simulink model "OpenLoop_2step"  (R2025a)
settings: Solver=ode4  StartTime=0.0  StopTime=5250  FixedStep=DT  MaxStep=DT  RelTol=1e-3  EnableMultiTasking=on
values from neighbouring files (symbols this model uses):
  particion = 301    [Run_OpenLoop_pr_2step.m]    (also in Run_OpenLoop_tl_2step.m)
  Ts = 0.025    [Run_OpenLoop_pr_2step.m]    (also in Run_OpenLoop_tl_2step.m)
  zona = 0.09    [Run_OpenLoop_pr_2step.m]    (also in Run_OpenLoop_tl_2step.m)
undefined symbols (not defined in the file or in its folder): DiscIntNeverNeededParam, OutList, strmatch
libraries: rllib x1
settings Model: Creator=bjonkman  LastModifiedBy=celop
settings SolverCC: AlgebraicLoopSolver=TrustRegion  AutoInsertRateTranBlk=on
settings DataIOCC: LimitDataPoints=on  SaveFormat=Array  SignalLoggingSaveFormat=ModelDataLogs  SaveOutput=off  SaveTime=off  SignalLoggingName=sigsOut
settings OptimizationCC: ExpressionDepthLimit=2147483647.0  LifeSpan=inf
settings DebuggingCC: SaveWithParameterizedLinksMsg=none  UnderspecifiedInitializationDetection=Classic  MergeDetectMultiDrivingBlocksExec=none  SignalResolutionControl=TryResolveAllWithWarning  MultiTaskDSMMsg=warning  MultiTaskCondExecSysMsg=none  FcnCallInpInsideContextMsg=warning  UnconnectedInputMsg=warning  UnconnectedOutputMsg=warning  UnconnectedLineMsg=warning  StateNameClashWarn=warning  SFUnexpectedBacktrackingDiag=warning  SFNoUnconditionalDefaultTransitionDiag=warning  SFExecutionAtInitializationDiag=none  ArithmeticOperatorsInVariantConditions=warning
settings HardwareCC: ProdBitPerPointer=32.0  ProdBitPerSizeT=32.0  ProdBitPerPtrDiffT=32.0  ProdLargestAtomicFloat=None  ProdIntDivRoundTo=Undefined  ProdEndianess=Unspecified  ProdWordSize=32.0  ProdHWDeviceType=32-bit Generic  TargetUnknown=on
settings ModelReferenceCC: EnableRefExpFcnMdlSchedulingChecks=on  PropagateSignalLabelsOutOfModel=off
settings SFSimCC: SimUseLocalCustomCode=off  CustomCodeUndefinedFunction=UseInterfaceOnly
settings RTWCC: RTWUseLocalCustomCode=off  GPUComputeCapability=3.5  DLArmComputeVersion=19.05
settings CodeAppCC: StateflowObjectComments=on
settings GRTTargetCC: TargetLangStandard=C89/C90 (ANSI)  CombineOutputUpdateFcns=off  GRTInterface=on
settings ConfigComp: CovMetricSettings=dw  CovSaveCumulativeToWorkspaceVar=on  CovSaveSingleToWorkspaceVar=on  CovExternalEMLEnable=off

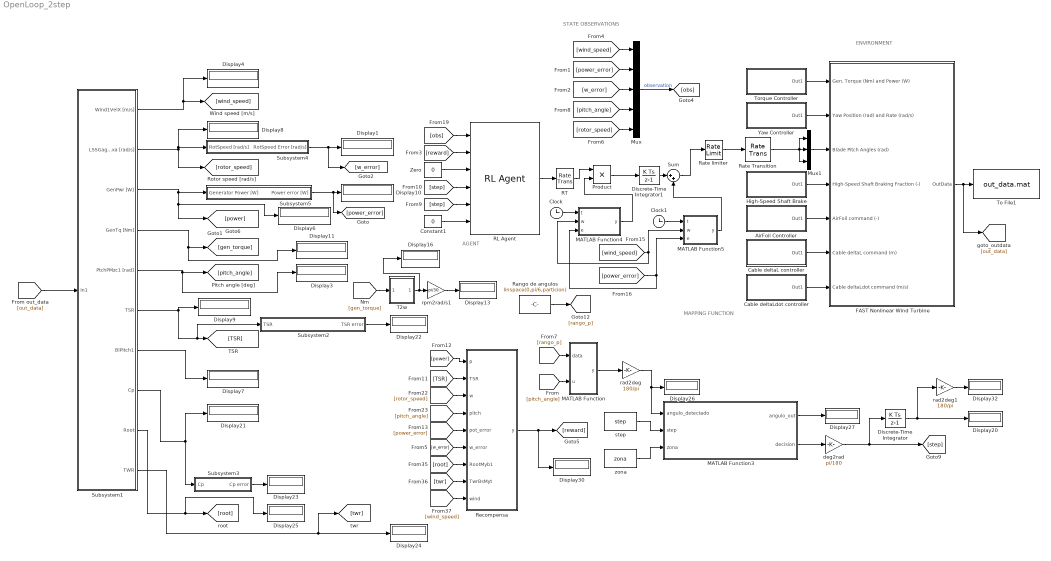
== system OpenLoop_2step ==
  note: STATE OBSERVATIONS
  note: AGENT
  note: ENVIRONMENT
  note: MAPPING FUNCTION
  AirFoil Controller : Subsystem
  Cable deltaL controller : Subsystem
  Cable deltaLdot controller : Subsystem
  Clock : Clock
  Clock1 : Clock
  Constant1 : Constant  Value=0
  Discrete-Time Integrator : DiscreteIntegrator  gainval=1.0/Ts  SampleTime=Ts  LimitOutput=on  UpperSaturationLimit=pi/6  LowerSaturationLimit=0  ICPrevOutput=DiscIntNeverNeededParam  ICPrevScaledInput=DiscIntNeverNeededParam
  Discrete-Time Integrator1 : DiscreteIntegrator  gainval=1.0/Ts  SampleTime=Ts  LimitOutput=on  UpperSaturationLimit=pi/6  LowerSaturationLimit=0  ICPrevOutput=DiscIntNeverNeededParam  ICPrevScaledInput=DiscIntNeverNeededParam
  Display{1,3..4,6..11,13,16,20..27,30,32} (21 alike) : Display
      Display30 settings: Format=short_e
  FAST Nonlinear Wind Turbine : Subsystem  mask(FAST Nonlinear Wind Turbine){}
      mask help: This block contains the FAST S-Function.
      mask init:
      | clear FAST_SFunc
  High-Speed Shaft Brake : Subsystem
  MATLAB Function : MATLAB Function  TreatAsAtomicUnit=on
  MATLAB Function3 : MATLAB Function  TreatAsAtomicUnit=on
  MATLAB Function4 : MATLAB Function  TreatAsAtomicUnit=on
  MATLAB Function5 : MATLAB Function  TreatAsAtomicUnit=on
  Mux : Mux  Inputs=5
  Mux1 : Mux  Inputs=3
  Product : Product
  RL Agent : rllib/RL Agent  Agent=agent  ExternalActionAsInput=on  ProvideLastAction=on  ProvideCumRwd=off  TreatAsDirectFeedthrough=on  UseStrictObservationDataTypes=off
  RT : RateTransition  OutPortSampleTime=0.025
  Rango de angulos : Constant  Value=linspace(0,pi/6,particion)
  Rate Transition : RateTransition  OutPortSampleTime=0.025
  Rate limiter : RateLimiter  RisingSlewLimit=7*pi/180  FallingSlewLimit=-7*pi/180  LinearizeAsGain=off
  Recompensa : MATLAB Function  TreatAsAtomicUnit=on
  Subsystem1 : Subsystem
  Subsystem2 : Subsystem
  Subsystem3 : Subsystem
  Subsystem4 : Subsystem
  Subsystem5 : Subsystem
  Sum : Sum  Inputs=|++
  T2w : Subsystem
  To File1 : ToFile  Filename=out_data.mat  MatrixName=data
  Torque Controller : Subsystem
  Yaw Controller : Subsystem
  Zero : Constant  Value=0  OutDataTypeStr=Inherit: Inherit via back propagation
  deg2rad : Gain  Gain=pi/180
  rad2deg : Gain  Gain=180/pi
  rad2deg1 : Gain  Gain=180/pi
  rpm2rad/s1 : Gain  Gain=pi/30
  step : Constant  Value=step
  zona : Constant  Value=zona
  wires:
  Yaw Controller/1(Out1) -> FAST Nonlinear Wind Turbine/2(Yaw Position (rad) and Rate (rad/s))
  High-Speed Shaft Brake/1(Out1) -> FAST Nonlinear Wind Turbine/4(High-Speed Shaft Braking Fraction (-))
  AirFoil Controller/1(Out1) -> FAST Nonlinear Wind Turbine/5(AirFoil command (-))
  Cable deltaL controller/1(Out1) -> FAST Nonlinear Wind Turbine/6(Cable deltaL command (m))
  Cable deltaLdot controller/1(Out1) -> FAST Nonlinear Wind Turbine/7(Cable deltaLdot command (m/s))
  Zero/1 -> RL Agent/3
  [rango_p] -> MATLAB Function/1(data)
  FAST Nonlinear Wind Turbine/1(OutData) -> To File1/1, [out_data]
  [out_data] -> Subsystem1/1(In1)
  Rate Transition/1 -> Mux1/3, Mux1/1, Mux1/2
  Constant1/1 -> RL Agent/6
  Subsystem1/3(GenPwr [W]) -> [power], Display6/1, Subsystem5/1(Generator Power [W])
  Subsystem1/1(Wind1VelX [m/s]) -> Display4/1, [wind_speed]
  Subsystem1/2(LSSGagVxa [rad/s]) -> Display8/1, Subsystem4/1(RotSpeed [rad/s]), [rotor_speed]
  [pitch_angle] -> MATLAB Function/2(u)
  [wind_speed] -> Mux/1
  MATLAB Function/1(y) -> rad2deg/1
  Subsystem1/5(PtchPMzc1 [rad]) -> Display3/1, [pitch_angle]
  Recompensa/1(y) -> Display30/1, [reward]
  [TSR] -> Recompensa/2(TSR)
  [pitch_angle] -> Recompensa/4(pitch)
  [rotor_speed] -> Recompensa/3(w)
  [power] -> Recompensa/1(p)
  Subsystem1/6(TSR) -> Display9/1, Subsystem2/1(TSR), [TSR]
  [power_error] -> Recompensa/5(pot_error)
  Subsystem1/7(BlPitch1) -> Display7/1
  [power_error] -> Mux/2
  [rotor_speed] -> Mux/5
  [pitch_angle] -> Mux/4
  [w_error] -> Mux/3
  [w_error] -> Recompensa/6(w_error)
  Rango de angulos/1 -> [rango_p]
  Subsystem5/1(Power error [W]) -> Display10/1, [power_error]
  Subsystem1/4(GenTq [Nm]) -> Display11/1, [gen_torque]
  Subsystem4/1(RotSpeed Error [rad/s]) -> Display1/1, [w_error]
  [gen_torque] -> T2w/1(In1)
  Mux/1 -> [obs]  "observation"
  [obs] -> RL Agent/1
  rpm2rad/s1/1 -> Display13/1
  T2w/1(Out1) -> Display16/1, rpm2rad/s1/1
  Subsystem2/1(TSR error) -> Display22/1
  Mux1/1 -> FAST Nonlinear Wind Turbine/3(Blade Pitch Angles (rad))
  Subsystem1/8(Cp) -> Subsystem3/1(Cp), Display21/1
  Subsystem3/1(Cp error) -> Display23/1
  [reward] -> RL Agent/2
  [root] -> Recompensa/7(RootMyb1)
  [twr] -> Recompensa/8(TwrBsMyt)
  Subsystem1/10(TWR) -> Display24/1, [twr]
  Subsystem1/9(Root) -> Display25/1, [root]
  rad2deg/1 -> Display26/1, MATLAB Function3/1(angulo_detectado)
  MATLAB Function3/1(angulo_out) -> Display27/1
  MATLAB Function3/2(decision) -> deg2rad/1
  [wind_speed] -> Recompensa/9(wind)
  Discrete-Time Integrator/1 -> rad2deg1/1, Display20/1
  rad2deg1/1 -> Display32/1
  [step] -> RL Agent/5
  [step] -> RL Agent/4
  deg2rad/1 -> [step], Discrete-Time Integrator/1
  step/1 -> MATLAB Function3/2(step)
  zona/1 -> MATLAB Function3/3(zona)
  Clock/1 -> MATLAB Function4/1(t)
  MATLAB Function4/1(y) -> Product/2
  [wind_speed] -> MATLAB Function4/2(w), MATLAB Function5/2(w)
  Product/1 -> Discrete-Time Integrator1/1
  RL Agent/1 -> RT/1
  Rate limiter/1 -> Rate Transition/1
  [power_error] -> MATLAB Function5/3(e), MATLAB Function4/3(e)
  RT/1 -> Product/1
  Discrete-Time Integrator1/1 -> Sum/1
  Sum/1 -> Rate limiter/1
  Clock1/1 -> MATLAB Function5/1(t)
  MATLAB Function5/1(y) -> Sum/2
  Torque Controller/1(Out1) -> FAST Nonlinear Wind Turbine/1(Gen. Torque (Nm) and Power (W))

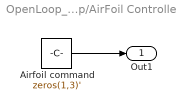
== system OpenLoop_2step/AirFoil Controller ==
  Airfoil command : Constant  Value=zeros(1,3)'
  Out1 : Outport
  wires:
  Airfoil command/1 -> Out1/1

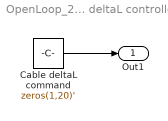
== system OpenLoop_2step/Cable deltaL controller ==
  Cable deltaL command : Constant  Value=zeros(1,20)'
  Out1 : Outport
  wires:
  Cable deltaL command/1 -> Out1/1

== system OpenLoop_2step/Cable deltaLdot controller ==
  Cable deltaLdot command : Constant  Value=zeros(1,20)'
  Out1 : Outport
  wires:
  Cable deltaLdot command/1 -> Out1/1

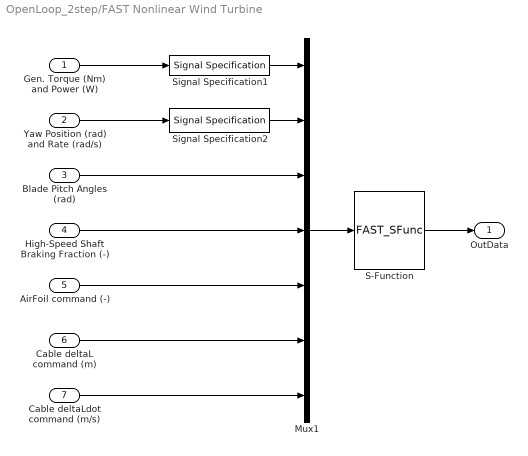
== system OpenLoop_2step/FAST Nonlinear Wind Turbine ==
  Gen. Torque (Nm) and Power (W) : Inport
  Yaw Position (rad) and Rate (rad/s) : Inport  Port=2
  Blade Pitch Angles (rad) : Inport  Port=3
  High-Speed Shaft Braking Fraction (-) : Inport  Port=4
  AirFoil command (-) : Inport  Port=5
  Cable deltaL command (m) : Inport  Port=6
  Cable deltaLdot command (m/s) : Inport  Port=7
  Mux1 : Mux  Inputs=7
  S-Function : S-Function  FunctionName=FAST_SFunc  Parameters=FAST_InputFileName, TMax, 0  SFunctionDeploymentMode=off  EnableBusSupport=off
  Signal Specification1 : SignalSpecification  OutDataTypeStr=double  Dimensions=2
  Signal Specification2 : SignalSpecification  OutDataTypeStr=double  Dimensions=2
  OutData : Outport
  wires:
  Gen. Torque (Nm) and Power (W)/1 -> Signal Specification1/1
  S-Function/1 -> OutData/1
  Mux1/1 -> S-Function/1
  Blade Pitch Angles (rad)/1 -> Mux1/3
  Yaw Position (rad) and Rate (rad/s)/1 -> Signal Specification2/1
  Signal Specification1/1 -> Mux1/1
  Signal Specification2/1 -> Mux1/2
  High-Speed Shaft Braking Fraction (-)/1 -> Mux1/4
  AirFoil command (-)/1 -> Mux1/5
  Cable deltaL command (m)/1 -> Mux1/6
  Cable deltaLdot command (m/s)/1 -> Mux1/7

== system OpenLoop_2step/High-Speed Shaft Brake ==
  High-Speed Shaft Braking Fraction : Constant  Value=0
  Out1 : Outport
  wires:
  High-Speed Shaft Braking Fraction/1 -> Out1/1

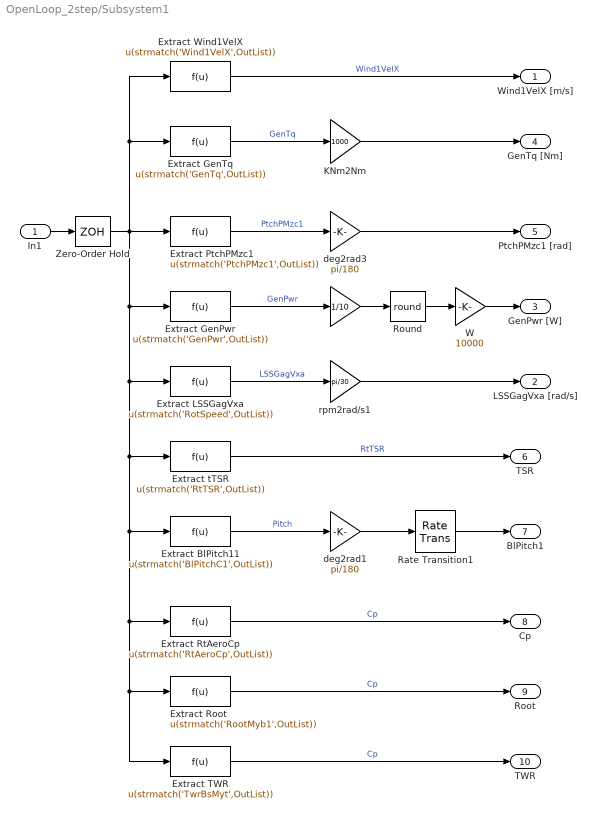
== system OpenLoop_2step/Subsystem1 ==
  In1 : Inport
  " " : Gain  Gain=1/10
  Extract BlPitch11 : Fcn  Expr=u(strmatch('BlPitchC1',OutList))
  Extract GenPwr : Fcn  Expr=u(strmatch('GenPwr',OutList))
  Extract GenTq : Fcn  Expr=u(strmatch('GenTq',OutList))
  Extract LSSGagVxa : Fcn  Expr=u(strmatch('RotSpeed',OutList))
  Extract PtchPMzc1 : Fcn  Expr=u(strmatch('PtchPMzc1',OutList))
  Extract Root : Fcn  Expr=u(strmatch('RootMyb1',OutList))
  Extract RtAeroCp : Fcn  Expr=u(strmatch('RtAeroCp',OutList))
  Extract TWR : Fcn  Expr=u(strmatch('TwrBsMyt',OutList))
  Extract Wind1VelX : Fcn  Expr=u(strmatch('Wind1VelX',OutList))
  Extract tTSR : Fcn  Expr=u(strmatch('RtTSR',OutList))
  KNm2Nm : Gain  Gain=1000
  Rate Transition1 : RateTransition  OutPortSampleTime=Ts
  Round : Rounding  Operator=round
  W : Gain  Gain=10000
  Zero-Order Hold : ZeroOrderHold  SampleTime=Ts
  deg2rad1 : Gain  Gain=pi/180
  deg2rad3 : Gain  Gain=pi/180
  rpm2rad/s1 : Gain  Gain=pi/30
  Wind1VelX [m/s] : Outport
  LSSGagVxa [rad/s] : Outport  Port=2
  GenPwr [W] : Outport  Port=3
  GenTq [Nm] : Outport  Port=4
  PtchPMzc1 [rad] : Outport  Port=5
  TSR : Outport  Port=6
  BlPitch1 : Outport  Port=7
  Cp : Outport  Port=8
  Root : Outport  Port=9
  TWR : Outport  Port=10
  wires:
  KNm2Nm/1 -> GenTq [Nm]/1
  Extract GenTq/1 -> KNm2Nm/1  "GenTq"
  Extract Wind1VelX/1 -> Wind1VelX [m/s]/1  "Wind1VelX"
  deg2rad3/1 -> PtchPMzc1 [rad]/1
  Extract PtchPMzc1/1 -> deg2rad3/1  "PtchPMzc1"
  Extract LSSGagVxa/1 -> rpm2rad/s1/1  "LSSGagVxa"
  Extract GenPwr/1 -> " "/1  "GenPwr"
  rpm2rad/s1/1 -> LSSGagVxa [rad/s]/1
  W/1 -> GenPwr [W]/1
  " "/1 -> Round/1
  Round/1 -> W/1
  In1/1 -> Zero-Order Hold/1
  Zero-Order Hold/1 -> Extract BlPitch11/1, Extract RtAeroCp/1, Extract Root/1, Extract TWR/1, Extract tTSR/1, Extract LSSGagVxa/1, Extract GenPwr/1, Extract GenTq/1, Extract Wind1VelX/1, Extract PtchPMzc1/1
  Extract tTSR/1 -> TSR/1  "RtTSR"
  Extract BlPitch11/1 -> deg2rad1/1  "Pitch"
  deg2rad1/1 -> Rate Transition1/1
  Rate Transition1/1 -> BlPitch1/1
  Extract RtAeroCp/1 -> Cp/1  "Cp"
  Extract TWR/1 -> TWR/1  "Cp"
  Extract Root/1 -> Root/1  "Cp"

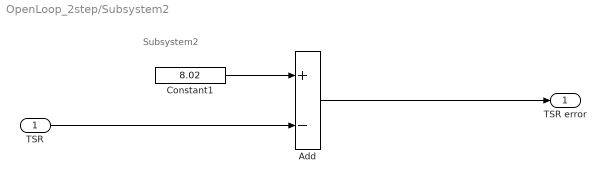
== system OpenLoop_2step/Subsystem2 ==
  note: Subsystem2
  TSR : Inport
  Add : Sum  Inputs=+-
  Constant1 : Constant  Value=8.02  SampleTime=Ts
  TSR error : Outport
  wires:
  Constant1/1 -> Add/1
  TSR/1 -> Add/2
  Add/1 -> TSR error/1

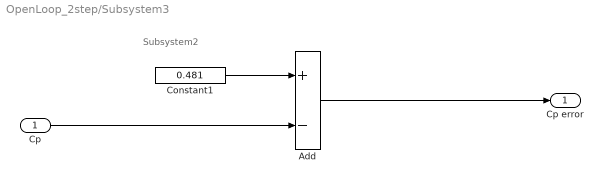
== system OpenLoop_2step/Subsystem3 ==
  note: Subsystem2
  Cp : Inport
  Add : Sum  Inputs=+-
  Constant1 : Constant  Value=0.481  SampleTime=Ts
  Cp error : Outport
  wires:
  Add/1 -> Cp error/1
  Cp/1 -> Add/2
  Constant1/1 -> Add/1

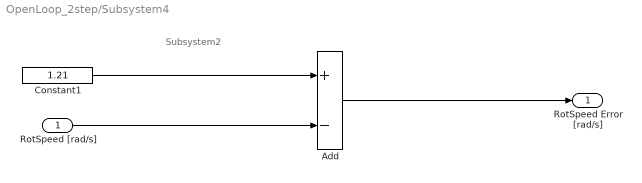
== system OpenLoop_2step/Subsystem4 ==
  note: Subsystem2
  RotSpeed [rad/s] : Inport
  Add : Sum  Inputs=+-
  Constant1 : Constant  Value=1.21  SampleTime=Ts
  RotSpeed Error [rad/s] : Outport
  wires:
  Add/1 -> RotSpeed Error [rad/s]/1
  RotSpeed [rad/s]/1 -> Add/2
  Constant1/1 -> Add/1

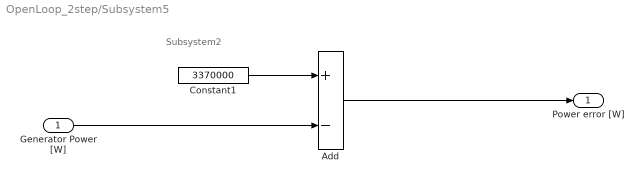
== system OpenLoop_2step/Subsystem5 ==
  note: Subsystem2
  Generator Power [W] : Inport
  Add : Sum  Inputs=+-
  Constant1 : Constant  Value=3370000  SampleTime=Ts
  Power error [W] : Outport
  wires:
  Add/1 -> Power error [W]/1
  Generator Power [W]/1 -> Add/2
  Constant1/1 -> Add/1

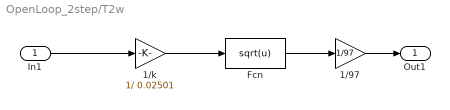
== system OpenLoop_2step/T2w ==
  In1 : Inport
  1/97 : Gain  Gain=1/97
  1/k : Gain  Gain=1/ 0.02501
  Fcn : Fcn  Expr=sqrt(u)
  Out1 : Outport
  wires:
  Fcn/1 -> 1/97/1
  1/k/1 -> Fcn/1
  1/97/1 -> Out1/1
  In1/1 -> 1/k/1

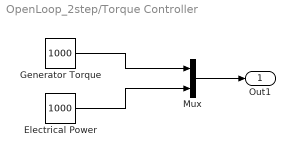
== system OpenLoop_2step/Torque Controller ==
  Electrical Power : Constant  Value=1000
  Generator Torque : Constant  Value=1000
  Mux : Mux  Inputs=2
  Out1 : Outport
  wires:
  Mux/1 -> Out1/1
  Generator Torque/1 -> Mux/1
  Electrical Power/1 -> Mux/2

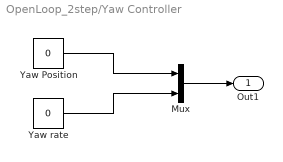
== system OpenLoop_2step/Yaw Controller ==
  Mux : Mux  Inputs=2
  Yaw Position : Constant  Value=0
  Yaw rate : Constant  Value=0
  Out1 : Outport
  wires:
  Mux/1 -> Out1/1
  Yaw Position/1 -> Mux/1
  Yaw rate/1 -> Mux/2

== matlab function OpenLoop_2step/MATLAB Function ==
  data: data input; u input; y output
function y = fcn(data, u)
if u>data(1) && u<data(end)
    y=data(discretize(u,data));
else
    if u<=data(1)
        y=data(1);
    else
        y=data(end);
    end
end

== matlab function OpenLoop_2step/Recompensa ==
  data: y output; p input; TSR input; w input; pitch input; pot_error input; w_error input; RootMyb1 input; TwrBsMyt input; wind input
function y = fcn(p,TSR, w,pitch,pot_error,w_error,RootMyb1 , TwrBsMyt, wind)
    % --- Constantes ---
    p_rated   = 3370000;     % [W]
    TSR_opt   = 8.02;
    w_rated = 1.21;
    omega_lim = [3 13]*pi/30;
    pitch_lim = [0 30]*pi/180;%0-30°
    TSR_lim = [3 9];
    % --- Limites de momentos ---
    M_root_max = 6000;   M_root_min = 0;   dM_root = M_root_max - M_root_min;%KNM
    M_twr_max  = 40000;  M_twr_min  = 0; dM_twr  = M_twr_max  - M_twr_min; %KNM
    
    % --- Recompensa ---
    if wind >= 9.5
        r_pow = 0.5*min(1,p / p_rated) + 0.5*min(1,w/w_rated);
    else
        r_pow = 1*min(1,TSR /  TSR_opt)   ; 
    end
    % --- Castigo por violar límites ---
    r_punishment = 0;
    
    if any([w<omega_lim(1), w>omega_lim(2), ...
             pitch<pitch_lim(1), pitch>pitch_lim(2), ...
        TSR<TSR_lim(1), TSR>TSR_lim(2)])
         r_punishment = -3;  
    end


    % Normalizar error respecto a la potencia nominal
   
    if wind >= 9.5
         r_error = -(abs(pot_error) / p_rated)^1 - (abs(w_error) / w_rated)^1;  % más negativo si el error es grande
    else
         r_error = -abs(TSR -  TSR_opt) /  TSR_opt;
    end    

    y = r_pow + r_punishment + r_error ;
end


    % 
    % exc_root = max(0, RootMyb1 - M_root_max)/dM_root + max(0, M_root_min - RootMyb1)/dM_root;
    % exc_twr  = max(0, TwrBsMyt - M_twr_max)/dM_twr  + max(0, M_twr_min - TwrBsMyt)/dM_twr;
    % r_root=-exc_root;
    % r_twr=-exc_twr;
% % --- Constantes ---
% p_rated   = 3370000;     % [W]
% TSR_rated   = 8.02;
% w_rated = 1.21;
% omega_lim = [3 13]*pi/30;
% pitch_lim = [0 30]*pi/180;%0-30°
% TSR_lim = [3 9];
% % --- Limites de momentos ---
% M_root_max = 6000;   M_root_min = 2000;   dM_root = M_root_max - M_root_min;%KNM
% M_twr_max  = 40000;  M_twr_min  = 20000; dM_twr  = M_twr_max  - M_twr_min; %KNM
% 
% % --- Recompensa ---
% r_pow = 0.5*min(1,p / p_rated) + 0.5*min(1,w/w_rated);
% 
% % --- Castigo por violar límites ---
% r_punishment = 0;
% 
% if any([w<omega_lim(1), w>omega_lim(2), ...
%          pitch<pitch_lim(1), pitch>pitch_lim(2), ...
%     TSR<TSR_lim(1), TSR>TSR_lim(2)])
%      r_punishment = -3;  
% end
% 
% % Normalizar error respecto a la potencia nominal
% r_error = -abs(pot_error) / p_rated - abs(w_error) / w_rated;  % más negativo si el error es grande
% 
% exc_root = max(0, RootMyb1 - M_root_max)/dM_root + max(0, M_root_min - RootMyb1)/dM_root;
% exc_twr  = max(0, TwrBsMyt - M_twr_max)/dM_twr  + max(0, M_twr_min - TwrBsMyt)/dM_twr;
% r_root=-exc_root;
% r_twr=-exc_twr;
% 
% 
% y = r_pow + r_punishment + r_error + 0*r_root;

== matlab function OpenLoop_2step/MATLAB Function4 ==
  data: t input; y output; w input; e input
function y = pitchrate(t,w,e)
% Pitch-rate scaling factor kappa_t.
% Nominal pitch rate = kappa * 0.4 deg/s (Delta_beta = 0.010 deg, Ts = 0.025 s).
%   t : simulation time [s]
%   w : hub-height wind speed [m/s] (unused)
%   e : power tracking error P_rated - P_out [W]
% --- Run settings (see README, Section 8) ----------------------------
    SAW10 = false;  % true only for the 10 m/s sawtooth profile
    MODE  = 1;      % 0 = fixed rate, 1 = two-level adaptive rule (0.8/0.3 deg/s)
    KFIX  = 1;      % fixed kappa (used only when MODE = 0)
% ---------------------------------------------------------------------
    % Start-up (excluded from the metrics, which use 200-5200 s)
    if SAW10
        if t < 50
            y = 1;  return      % 0.4 deg/s
        end
    else
        if t < 10
            y = 10;  return     % 4 deg/s
        elseif t < 15
            y = 5;   return     % 2 deg/s
        elseif t < 200
            y = 2.5; return     % 1 deg/s
        end
    end
    % Configuración evaluada
    if MODE == 1
        if abs(e) > 0.1e6
            y = 2;      % 0.8 deg/s
        else
            y = 0.75;   % 0.3 deg/s
        end
    else
        y = KFIX;
    end
end

== matlab function OpenLoop_2step/MATLAB Function3 ==
  data: angulo_detectado input; angulo_out output; decision output; step input; zona input
function [angulo_out, decision] = logica_seguimiento(angulo_detectado,step,zona)
    % CONFIGURACIÓN
    paso = step;% Cuánto incrementa/decrementa

    zona_muerta = zona;   % Tolerancia para considerar que son iguales
    angulo_inicial = 0;  % Valor de arranque

    % ESTADO (Memoria)
    persistent angulo_interno;

    % Inicialización en la primera ejecución
    if isempty(angulo_interno)
        angulo_interno = angulo_inicial;
    end

    % CÁLCULO DEL ERROR
    error = angulo_detectado - angulo_interno;

    % LÓGICA DE DECISIÓN
    % decision = 1  -> Incrementa
    % decision = -1 -> Decrementa
    % decision = 0  -> Mantiene (Igualdad)

    if error > zona_muerta
        decision = paso;
        angulo_interno = angulo_interno + paso;

    elseif error < -zona_muerta
        decision = -paso;
        angulo_interno = angulo_interno - paso;

    else
        decision = 0;
        % No cambiamos el angulo_interno
    end

    % ASIGNACIÓN DE SALIDAS
    angulo_out = angulo_interno;
end

== matlab function OpenLoop_2step/MATLAB Function5 ==
  data: t input; y output; w input; e input
function y = offset(t,w,e)
% Pitch offset for the diagnostic test of the transition profile (Section 6.2).
%   t : simulation time [s]
%   w : hub-height wind speed [m/s]
%   e : power tracking error [W] (unused)
% Default: no offset (k = 0), used for all results except the diagnostic test.
% Diagnostic test (10 m/s sawtooth, kappa = 0.01):
%   k = -1*pi/180 for t > 51 s and w < 9.8 m/s (rated wind speed).
    if t < 10
        k = 0;     
    elseif t < 15
        k = 0;     
    elseif t < 51
        k = 0;    
    elseif t > 51 && w < 9.8
        k = 0*pi/180 ; %-1*pi/180;
    else
        k = 0*pi/180 ;
    end
    y = k;
end
